simulink model "simulink13"  (R2021b)
settings: Solver=VariableStepAuto  StartTime=0.0  StopTime=100.0  RelTol=1e-3
settings Model: Creator=13676840  LastModifiedBy=13676840

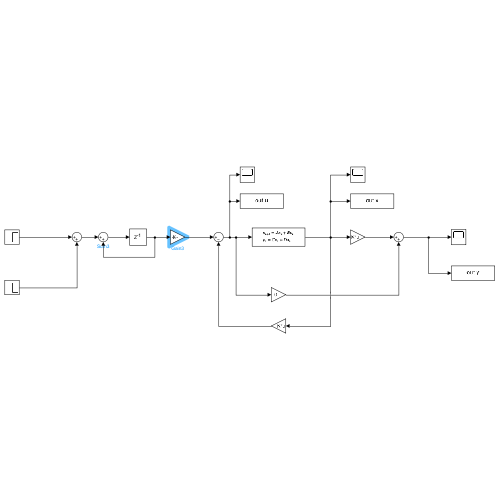
[thumbnail: Simulink's stored preview of the top-level diagram]
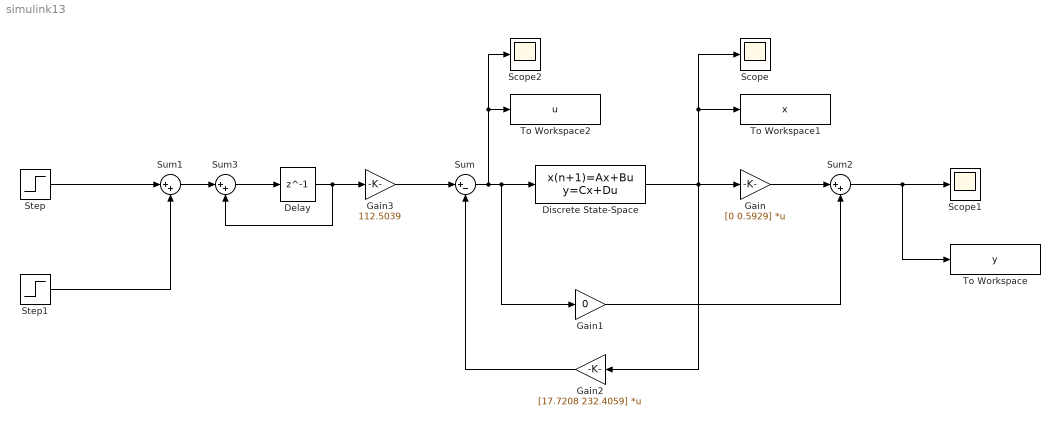
== system simulink13 ==
  Delay : Delay  DelayLength=1  InitialCondition=0
  Discrete State-Space : DiscreteStateSpace  A=[0.8672 -0.0496; 0.0836 0.9977]  B=[0.0836; 0.0038]  C=[1 0; 0 1]  D=[0; 0]  SampleTime=0.2241
  Gain : Gain  Gain=[0 0.5929]  Multiplication=Matrix(K*u)
  Gain1 : Gain  Gain=0
  Gain2 : Gain  Gain=[17.7208 232.4059]  Multiplication=Matrix(K*u)
  Gain3 : Gain  Gain=112.5039
  Scope : Scope
  Scope1 : Scope
  Scope2 : Scope
  Step : Step  Time=0  After=1.17  SampleTime=0
  Step1 : Step  Time=12  After=-0.15  SampleTime=0
  Sum : Sum  Inputs=|+-
  Sum1 : Sum  Inputs=|++
  Sum2 : Sum  Inputs=|++
  Sum3 : Sum  Inputs=|++
  To Workspace : ToWorkspace  VariableName=y  SaveFormat=Timeseries  SampleTime=-1
  To Workspace1 : ToWorkspace  VariableName=x  SaveFormat=Timeseries  SampleTime=-1
  To Workspace2 : ToWorkspace  VariableName=u  SaveFormat=Timeseries  SampleTime=-1
  wires:
  Step/1 -> Sum1/1
  Step1/1 -> Sum1/2
  Sum/1 -> To Workspace2/1, Scope2/1, Gain1/1, Discrete State-Space/1
  Gain2/1 -> Sum/2
  Discrete State-Space/1 -> Scope/1, To Workspace1/1, Gain2/1, Gain/1
  Gain/1 -> Sum2/1
  Sum2/1 -> To Workspace/1, Scope1/1
  Gain1/1 -> Sum2/2
  Sum1/1 -> Sum3/1
  Sum3/1 -> Delay/1
  Delay/1 -> Sum3/2, Gain3/1
  Gain3/1 -> Sum/1
